simulink model "Bench_ISCS"  (R2026b)
settings: Solver=ode1  StopTime=T_end  FixedStep=Ts
undefined symbols (not defined in the file): du_min, ISCS_Ad, ISCS_Bd, ISCS_Cd, ISCS_Dd, ISCS_Tu, ISCS_Ty, Ts
settings Model: Creator=williamvandevoir  LastModifiedBy=williamvandevoir

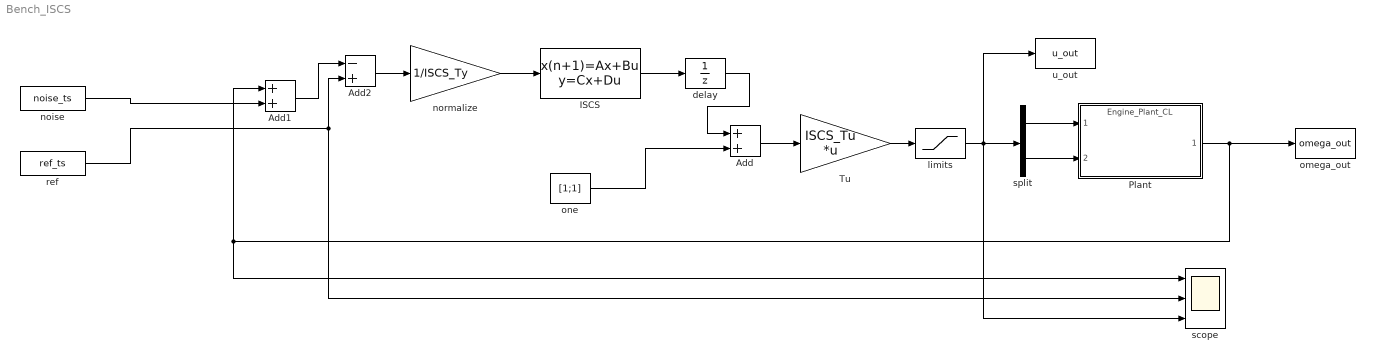
== system Bench_ISCS ==
  Add : Sum
  Add1 : Sum
  Add2 : Sum  Inputs=-+
  ISCS : DiscreteStateSpace  A=ISCS_Ad  B=ISCS_Bd  C=ISCS_Cd  D=ISCS_Dd  InitialCondition=zeros(12,1)  SampleTime=Ts
  Plant : ModelReference  ModelNameDialog=Engine_Plant_CL  SimulationMode=Normal  ModelReferenceVersion=1.23
  Tu : Gain  Gain=ISCS_Tu  Multiplication=Matrix(K*u)
  delay : UnitDelay  InitialCondition=zeros(2,1)  SampleTime=Ts
  limits : Saturate  UpperLimit=[100; 0]  LowerLimit=[0; du_min]
  noise : FromWorkspace  VariableName=noise_ts  Interpolate=off  OutputAfterFinalValue=Holding final value
  normalize : Gain  Gain=1/ISCS_Ty
  omega_out : ToWorkspace  VariableName=omega_out  SaveFormat=Timeseries  SampleTime=-1
  one : Constant  Value=[1;1]
  ref : FromWorkspace  VariableName=ref_ts  Interpolate=off  OutputAfterFinalValue=Holding final value
  scope : Scope  NumInputPorts=3
  split : Demux  Outputs=2
  u_out : ToWorkspace  VariableName=u_out  SaveFormat=Timeseries  SampleTime=-1
  wires:
  limits/1 -> split/1, scope/3, u_out/1
  Tu/1 -> limits/1
  delay/1 -> Add/1
  ISCS/1 -> delay/1
  normalize/1 -> ISCS/1
  Plant/1 -> omega_out/1, Add1/1, scope/1
  Add2/1 -> normalize/1
  Add/1 -> Tu/1
  split/2 -> Plant/2
  ref/1 -> Add2/2, scope/2
  Add1/1 -> Add2/1
  split/1 -> Plant/1
  one/1 -> Add/2
  noise/1 -> Add1/2
